simulink model "CurrentSense"  (R2026b)
settings: Solver=VariableStepAuto
values from neighbouring files (symbols this model uses):
  Cur_AdcFullScale = 1023    [DCMotorParams.m]
  Cur_AdcVref = 5    [DCMotorParams.m]
  Cur_FilterCoef = 0.2    [DCMotorParams.m]
  Cur_Offset_V = 3.54    [DCMotorParams.m]
  Cur_Sensitivity = 0.185    [DCMotorParams.m]
  Ts = 0.01    [DCMotorParams.m]
libraries: arduinolib x1
settings Model: Creator=bence  LastModifiedBy=bence

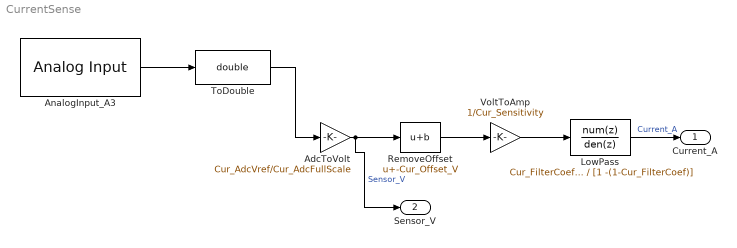
== system CurrentSense ==
  AdcToVolt : Gain  Gain=Cur_AdcVref/Cur_AdcFullScale
  AnalogInput_A3 : arduinolib/Analog Input  pinNumber=Cur_AdcPin  ReadResultsOnly=off  ConversionTriggerSource=Software  ExternalTriggerType=uint32( 0 )  OutputDataType=uint16  EnableConversionCompleteNotify=off  EnableOuputStatus=off  SampleTime=Ts  blockPlatform=arduino
  LowPass : DiscreteFilter  Numerator=Cur_FilterCoef  Denominator=[1 -(1-Cur_FilterCoef)]
  RemoveOffset : Bias  Bias=-Cur_Offset_V  SaturateOnIntegerOverflow=off
  ToDouble : DataTypeConversion  OutDataTypeStr=double  SaturateOnIntegerOverflow=off  RndMeth=Floor
  VoltToAmp : Gain  Gain=1/Cur_Sensitivity
  Current_A : Outport
  Sensor_V : Outport  Port=2
  wires:
  AnalogInput_A3/1 -> ToDouble/1
  RemoveOffset/1 -> VoltToAmp/1
  VoltToAmp/1 -> LowPass/1
  LowPass/1 -> Current_A/1  "Current_A"
  ToDouble/1 -> AdcToVolt/1
  AdcToVolt/1 -> RemoveOffset/1, Sensor_V/1  "Sensor_V"
